simulink model "PSO_BON"  (R2019b)
settings: Solver=VariableStepAuto  StartTime=0.0  StopTime=0.2  RelTol=1e-5
undefined symbols (not defined in the file): sigbuilder_block
libraries: powerlib x164, re_lib x96, powerlib_meascontrol x9
(part 6 of 6)

== matlab function PSO_BON/Variant PSO/MATLAB Function1 ==
  settings: updateMethod=DISCRETE  sampleTime=1e-4
  data: Vpv input; Duty output; Ipv input
function Duty = PSO_SSR(Vpv,Ipv)
coder.extrinsic('rand')
coder.extrinsic('format long')

persistent Npart_3 v_3 iter_3 count_Part_3 count_3 pos_3 fitness_3 fitnessPbest_3 Pbest_3 fitnessGbest_3 fitnessGworst_3 Gbest_3 Gworst_3 count_conv_3 reinit_3 Duty_Init_3;
maxiter = 10000000;                                                         % Nombre d'itération

% Définition de l'espace de recherche
% ------------------------------------
duty_cl_min = 0.1;                                                          % Valeur minimale du rapport cyclique
duty_cl_max = 0.9;                                                          % Valeur maximale du rapport cyclique

% Tolérance de la puissance
% ------------------------------------
tolerance = 0.01;                                                           % Tolerance de la puissance en sortie

% Initialisation des vitesses des particules
% -------------------------------------------
if(isempty(Npart_3))
    Npart_3 = 10;
end
if(isempty(v_3))
    v_3 = zeros(Npart_3,1);
end

% Initialisation des positions des particules
% -------------------------------------------

% hybrid initialisation
% ---------------------  
if(isempty(pos_3))                                                          % Si la position des particules est inexistant
    r = zeros(Npart_3,1);
    r = rand(Npart_3,1);
    pos_3 = zeros(Npart_3,1);
    for i = 1:Npart_3-2
        Min = duty_cl_min + (i-1)*(duty_cl_max-duty_cl_min)/(Npart_3-2);
        Max = Min + (duty_cl_max-duty_cl_min)/(Npart_3-2);
        pos_3(i+1) = Min + r(i)*(Max-Min);
    end
    pos_3(1) = duty_cl_min;
    pos_3(Npart_3) = duty_cl_max;
end

% % Uniform initialisation
% % ----------------------  
% if(isempty(pos_3))                                                          % Si la position des particules est inexistant
%     pos_3 = zeros(Npart_3,1);
%     for i = 1:Npart_3-2
%         pos_3(i+1) = duty_cl_min + ((duty_cl_max-duty_cl_min)*(i-1))/(Npart_3-1);
%     end
%     pos_3(1) = duty_cl_min;
%     pos_3(Npart_3) = duty_cl_max;
% end
% 
% % Random initialisation
% % ---------------------  
% if(isempty(pos_3))                                                          % Si la position des particules est inexistant
%     pos_3 = zeros(Npart_3,1);
%     for i = 1:Npart_3-2
%         pos_3(i+1) = duty_cl_min + rand(1)*(duty_cl_max-duty_cl_min);
%     end
%     pos_3(1) = duty_cl_min;
%     pos_3(Npart_3) = duty_cl_max;
% end

% pos
% Initialisation des parametres persitents
% -------------------------------------------------
if(isempty(iter_3))       % Si le numéro de l'iteration est inexistant fixe à 1
    iter_3 = 1;
end
if(isempty(fitness_3))    % Si la fonction cout des particules est inexistant
    fitness_3 = zeros(Npart_3,1);
end
if(isempty(fitnessPbest_3))   % Si les fonctions couts des meilleures positions des particules est inexistant
    fitnessPbest_3 = zeros(Npart_3,1);
end
if(isempty(Pbest_3))      % Si les meilleures positions des particules est inexistant
    Pbest_3 = zeros(Npart_3,1);
end
if(isempty(Gbest_3))      % Si la meilleure position de l'éssain est inexistant
    Gbest_3 = zeros(maxiter,1);
end
if(isempty(Gworst_3))      % Si la meilleure position de l'éssain est inexistant
    Gworst_3 = zeros(maxiter,1);
end
if(isempty(fitnessGbest_3))   % Si la fonction cout de la meilleure position de l'éssain est inexistant
    fitnessGbest_3 = zeros(maxiter,1);
end
if(isempty(fitnessGworst_3))   % Si la fonction cout de la meilleure position de l'éssain est inexistant
    fitnessGworst_3 = zeros(maxiter,1);
end
if(isempty(count_Part_3)) % Si le compteur de particule est inexistant
    count_Part_3 = 1;
end
if(isempty(count_conv_3)) % Si le compteur de particule convergente est inexistant
    count_conv_3 = zeros(Npart_3,1);
end
if(isempty(reinit_3))   % Si le coefficeint de reinitialisation est inexistant
    reinit_3 = 0;
end
if(isempty(Duty_Init_3))
    Duty_Init_3 = 0;
end
if(isempty(count_3))      % Si le compteur du régime transitoire est inexistant
    count_3 = 1;
end


% Evaluation des particules initiales
% -------------------------------------------------

%% phase transitoire d'évaluation d'une particule
% -------------------------------------------------
if (count_3 >= 1 && count_3 <= 20)
    Duty = pos_3(count_Part_3);
    count_3 = count_3 + 1;

    %% En cas de convergence
    % ---------------------------------------------
    if (reinit_3 == 1)  
        fitnessGbest_3(iter_3) = Vpv*Ipv;
        Duty = Duty_Init_3;
            if (abs(fitnessGbest_3(iter_3) - fitnessGbest_3(iter_3-1)) < 1)
                count_3 = count_3 - 1;
                reinit_3 = 1;
            else
                reinit_3 = 0;
                Npart_3 = 10;
                r = zeros(Npart_3,1);
                r = rand(Npart_3,1);
                pos_3 = zeros(Npart_3,1);
                for i = 1:Npart_3-2
                    Min = duty_cl_min + (i-1)*(duty_cl_max-duty_cl_min)/(Npart_3-2);
                    Max = Min + (duty_cl_max-duty_cl_min)/(Npart_3-2);
                    pos_3(i+1) = Min + r(i)*(Max-Min);
                end
                pos_3(1) = duty_cl_min;
                pos_3(Npart_3) = duty_cl_max;
                iter_3 = 0;
                v_3 = zeros(Npart_3,1);
                fitness_3 = zeros(Npart_3,1);
                fitnessPbest_3 = zeros(Npart_3,1);
                Pbest_3 = zeros(Npart_3,1);
                Gbest_3 = zeros(maxiter,1);
                Gworst_3 = zeros(maxiter,1);
                fitnessGbest_3 = zeros(maxiter,1);
                fitnessGworst_3 = zeros(maxiter,1);
                count_Part_3 = 1;
                count_conv_3 = zeros(Npart_3,1);
                Duty_Init_3 = 0;
                count_3 = 1;
                iter_3 = iter_3 + 1;
            end 
    end
    return;
    
%%
Npart_3;
count_Part_3;
else
    Npart_3
    count_Part_3
    if(count_Part_3 <= (Npart_3 - 1))
        Duty = pos_3(count_Part_3 + 1);
    else
        Duty = pos_3(1);
    end
end
iter_3;
% pos
% fitness
% fitnessPbest

                        % Programme PSO principale ou se fait la
                        % mise à jour des Pbest, de Gbest, des vitesse et
                        % des positions des particules
                        % -------------------------------------------------
fitness_3(count_Part_3) = Vpv*Ipv;  % Fonction cout des particules
if (count_Part_3 <= (Npart_3 - 1))
    count_Part_3 = count_Part_3 + 1;
    count_3 = 2;
else
    nnn = 1;
    if (iter_3 == 1)
                        % Initialisation des Pbest
                        % -------------------------------------------------
            for i = 1:Npart_3
                Pbest_3(i) = pos_3(i);
                fitnessPbest_3(i) = fitness_3(i);
            end
                        % Détermination de la fonction cout maximale
                        % -------------------------------------------------
        maxFitnessPbest = 0;
        for j = 1:length(fitnessPbest_3)
            if fitnessPbest_3(j) > maxFitnessPbest
                maxFitnessPbest = fitnessPbest_3(j);
            end
        end
                        % Initialisation de Gbest
                        % -------------------------------------------------
        fitnessGbest_3(iter_3) = maxFitnessPbest;
            for k = 1:Npart_3
                if(fitnessGbest_3(iter_3) == fitnessPbest_3(k))
                    Gbest_3(iter_3) = Pbest_3(k);
                end
            end
    elseif (iter_3 >= 2 && iter_3 <= maxiter)
                        % Mise à jour des Pbest
                        % -------------------------------------------------
            for i = 1:Npart_3
                if (fitness_3(i) > fitnessPbest_3(i))
                    Pbest_3(i) = pos_3(i);
                    fitnessPbest_3(i) = fitness_3(i);
                end
            end
                        % Mise à jour de Gbest
                        % -------------------------------------------------
        maxFitnessPbest = 0;
        minFitnessPbest = 100000;
        for j = 1:length(fitnessPbest_3)
            if fitnessPbest_3(j) > maxFitnessPbest
                maxFitnessPbest = fitnessPbest_3(j);
            end
            if fitnessPbest_3(j) < minFitnessPbest
                minFitnessPbest = fitnessPbest_3(j);
            end
        end
        fitnessGbest_3(iter_3) = maxFitnessPbest;
        fitnessGworst_3(iter_3) = minFitnessPbest;
            nn = 0;
            for k=1:Npart_3
                if(fitnessGbest_3(iter_3) == fitnessPbest_3(k))
                    Gbest_3(iter_3) = Pbest_3(k);
                end
                if(fitnessGworst_3(iter_3) == fitnessPbest_3(k))
                    Gworst_3(iter_3) = Pbest_3(k);
                    nn = k;
                end
            end
        nn;
        if (iter_3 > 2)
            if (Npart_3 >= 2)
                Npart_3 = Npart_3 - nnn;
                Pbest_3(nn) = [];
                pos_3(nn) = [];
                fitness_3(nn) = [];
                fitnessPbest_3(nn) = [];
                v_3(nn) = [];
                count_conv_3(nn) = [];
                nnn = nnn + 1;
            end
        end
    end
    pos_3;
    count_Part_3;
    iter_3;
    Npart_3
    count_Part_3
                        % Test de convergence
                        % -------------------------------------------------
        for i = 1:Npart_3
            if ((fitnessGbest_3(iter_3) - fitnessPbest_3(i)) < tolerance)
                if ((Gbest_3(iter_3) - pos_3(i)) < 0.0001)
                    count_conv_3(i) = 1;
                end
            end
        end
    n = sum(count_conv_3);
    if (n == Npart_3)
        reinit_3 = 1;
        Duty_Init_3 = Gbest_3(iter_3);
    else
        count_conv_3 = zeros(Npart_3,1);
    end
                        % Mise à jour des positions et des vitesses des
                        % particules
                        % -------------------------------------------------
        for i = 1:Npart_3
            v_3(i) = updatevelocity(v_3(i),Pbest_3(i),pos_3(i),Gbest_3(iter_3),iter_3,50);
            pos_3(i) = updateduty(pos_3(i),v_3(i));
            if (pos_3(i) > duty_cl_max)
                pos_3(i) = duty_cl_max;
            end
            if (pos_3(i) < duty_cl_min)
                pos_3(i) = duty_cl_min;
            end
        end
                        % Mise à jour des positions et des vitesses
                        % -------------------------------------------------

                        % Contraindre la position mise à jour dans
                        % l'intervale de recherche
                        % -------------------------------------------------
    Duty = pos_3(1);
    count_Part_3 = 1;
    count_3 = 2;
    iter_3 = iter_3 + 1;
    if iter_3 > maxiter
        iter_3 = maxiter;
    end
end
end

function vfinal=updatevelocity(velocity,pobest,d,gwbest,Iter, Maxiter)

w1 = 0.1;
w2 = 0.2;
w = ((w1 - w2)*(Maxiter - Iter))/Maxiter + w2;

c1f = 0.0015;       % Personal Learning Coefficient
c1i = 1;         % Global Learning Coefficient
c1 = ((c1f - c1i)*(Iter))/Maxiter + c1i;

c2f = 1.4;       % Personal Learning Coefficient
c2i = 0.3;         % Global Learning Coefficient
c2 = ((c2f - c2i)*(Iter))/Maxiter + c2i;

vfinal = (w*velocity)+(c1*rand(1)*(pobest-d))+(c2*rand(1)*(gwbest-d));
% vfinal = (w*velocity)+beta*(gwbest-d);
end
function dfinal=updateduty(d,velocity)
dup=d+velocity;
if(dup>0.9)
    dfinal=0.9;
elseif(dup<0.1)
    dfinal=0.1;
else
    dfinal=dup;
end
end

== matlab function PSO_BON/Dynamique PSOO/MATLAB Function1 ==
  settings: updateMethod=DISCRETE  sampleTime=1e-4
  data: Vpv input; D output; Ipv input
function D = PSO(Vpv,Ipv)
%#codegen
persistent u;
persistent dcurrent;
persistent pbest;
persistent p;
persistent dc;
persistent v;
persistent counter;
persistent gbest;
persistent K;
Npart = 10;
maxIte = 15;
if(isempty(counter))
    counter=0;
end
if(isempty(dcurrent))
    dcurrent=0.5;
end
if(isempty(gbest))
    gbest=0.5;
end
if(isempty(p))
    p=zeros(Npart,1);
end
if(isempty(K))
    K=0;
end
if(isempty(v))
    v=zeros(Npart,1);
end

if(isempty(pbest))
    pbest=zeros(Npart,1);
end
if(isempty(u))
    u=0;
end
if(isempty(dc))
    dc=zeros(Npart,1);
    dc(1)=0;
    dc(2)=0.1;
    dc(3)=0.2;
    dc(4)=0.3;
    dc(5)=0.4;
    dc(6)=0.5;
    dc(7)=0.6;
    dc(8)=0.7;
    dc(9)=0.8;
    dc(10)=0.9;
end
if(counter>=1 && counter<20)
    D=dcurrent;
    counter=counter+1;
    return;
end
counter=0;

if(u>=1 && u<=Npart)
    if((Vpv*Ipv)>p(u))
        p(u)=Vpv*Ipv;
        pbest(u)=dcurrent;
    end
end
u=u+1;
if(u==Npart+2)
    u=1;
end
if(u==1)
    D=dc(u);
    dcurrent=D;
    counter=1;
    return;
elseif(u==2)
    D=dc(u);
    dcurrent=D;
    counter=1;
    return;
elseif(u==3)
    D=dc(u);
    dcurrent=D;
    counter=1;
    return;
elseif(u==4)
    D=dc(u);
    dcurrent=D;
    counter=1;
    return;
elseif(u==5)
    D=dc(u);
    dcurrent=D;
    counter=1;
    return;
elseif(u==6)
    D=dc(u);
    dcurrent=D;
    counter=1;
    return;
elseif(u==7)
    D=dc(u);
    dcurrent=D;
    counter=1;
    return;
elseif(u==8)
    D=dc(u);
    dcurrent=D;
    counter=1;
    return;
elseif(u==9)
    D=dc(u);
    dcurrent=D;
    counter=1;
    return;
elseif(u==10)
    D=dc(u);
    dcurrent=D;
    counter=1;
    return;
elseif(u==Npart+1)
    [m,i]=max(p);
    gbest=pbest(i);
    D=gbest;
    dcurrent=D;
    counter=1;
    K = K + 1;
    %update velocity and duty cycle
    v(1)=updatevelocity(v(1),pbest(1),dc(1),gbest,maxIte,K)
    v(2)=updatevelocity(v(2),pbest(2),dc(2),gbest,maxIte,K)
    v(3)=updatevelocity(v(3),pbest(3),dc(3),gbest,maxIte,K)
    v(4)=updatevelocity(v(4),pbest(4),dc(4),gbest,maxIte,K)
    v(5)=updatevelocity(v(5),pbest(5),dc(5),gbest,maxIte,K)
    v(6)=updatevelocity(v(6),pbest(6),dc(6),gbest,maxIte,K)
    v(7)=updatevelocity(v(7),pbest(7),dc(7),gbest,maxIte,K)
    v(8)=updatevelocity(v(8),pbest(8),dc(8),gbest,maxIte,K)
    v(9)=updatevelocity(v(9),pbest(9),dc(9),gbest,maxIte,K)
    v(10)=updatevelocity(v(10),pbest(10),dc(10),gbest,maxIte,K)
    %update duty cycle
    dc(1)=updateduty(dc(1),v(1))
    dc(2)=updateduty(dc(2),v(2))
    dc(3)=updateduty(dc(3),v(3))
    dc(4)=updateduty(dc(4),v(4))
    dc(5)=updateduty(dc(5),v(5))
    dc(6)=updateduty(dc(6),v(6))
    dc(7)=updateduty(dc(7),v(7))
    dc(8)=updateduty(dc(8),v(8))
    dc(9)=updateduty(dc(9),v(9))
    dc(10)=updateduty(dc(10),v(10))
    
    return;
    
else
    u
    y='hello'
    D=0.1
    
end


end
function vfinal=updatevelocity(velocity,pobest,d,gwbest,maxIte,K)
% PSO Parameters
w=0.4;
c1=1.2;       % Personal Learning Coefficient
c2=2;         % Global Learning Coefficient
beta = 1.5;
wmax=1; wmin=0.1; %w=0.5; 
c1max=1.2;  c1min=1; c2max=1.6;  c2min=1;
w=wmax-(wmax-wmin)/maxIte*K;
c1=c1max-(c1max-c1min)/maxIte*K;
c2=c2max-(c2max-c2min)/maxIte*K;
% % Constriction Coefficients
% phi1=2.05;
% phi2=2.05;
% phi=phi1+phi2;
% chi=2/(phi-2+sqrt(phi^2-4*phi));
% w=chi;          % Inertia Weight
% wdamp=1;        % Inertia Weight Damping Ratio
% c1=chi*phi1;    % Personal Learning Coefficient
% c2=chi*phi2;    % Global Learning Coefficient
vfinal = (w*velocity)+(c1*rand(1)*(pobest-d))+(c2*rand(1)*(gwbest-d));
% vfinal = (w*velocity)+beta*(gwbest-d);
end
function dfinal=updateduty(d,velocity)
dup=d+velocity;
if(dup>0.9)
    dfinal=0.9;
elseif(dup<0.1)
    dfinal=0.1;
else
    dfinal=dup;
end
end

== matlab function PSO_BON/P&O/MATLAB Function1 ==
  settings: updateMethod=DISCRETE  sampleTime=1e-4
  data: Vpv input; D output; Ipv input
function D = PSO_Mod(Vpv,Ipv)
coder.extrinsic('rand')
coder.extrinsic('format long')

persistent iter count_Part count pos fitness fitnessPbest Pbest fitnessGbest Gbest count_conv reinit Duty_Init Vpos Ipos;
persistent Vgbest Igbest Vposbest Iposbest;
Npart = 5;              % Nombre de particules de l'éssain
maxiter = 10000000;           % Nombre d'itération
delta = 0.05;
% Espace de recherche
% ------------------------------------
duty_cl_min = 0.1;      % Valeur minimale du rapport cyclique
duty_cl_max = 0.9;      % Valeur maximale du rapport cyclique

% Tolérance de la puissance
% ------------------------------------
tolerance = 1;          % Tolerance de la puissance en sortie

% Initialisation des positions des particules
% ------------------------------------
r = zeros(Npart,1);     % génération d'un vecteur de nombre aléatoire compris entre 0 et 1
r = rand(Npart,1);      
if(isempty(pos))        % Si la position des particules est inexistant
    pos = zeros(Npart,1);
%     for i = 1:Npart
%         pos(i) = duty_cl_min + ((duty_cl_max-duty_cl_min)*(i-1))/(Npart-1);
% %         pos(i) = duty_cl_min + r(i)*(duty_cl_max-duty_cl_min);
%     end
    
    for i = 1:Npart-2
        Min = duty_cl_min + (i-1)*(duty_cl_max-duty_cl_min)/(Npart-2);
        Max = Min + (duty_cl_max-duty_cl_min)/(Npart-2);
        pos(i+1) = Min + r(i)*(Max-Min);
    end
    pos(1) = duty_cl_min;
    pos(Npart) = duty_cl_max;
    Pp = pos;
end

% Initialisation des parametres persitents
% -------------------------------------------------
if(isempty(iter))       % Si le numéro de l'iteration est inexistant fixe à 1
    iter = 1;
end
if(isempty(fitness))    % Si la fonction cout des particules est inexistant
    fitness = zeros(Npart,1);
end
if(isempty(Vpos))    % Si la fonction cout des particules est inexistant
    Vpos = zeros(Npart,1);
end
if(isempty(Ipos))    % Si la fonction cout des particules est inexistant
    Ipos = zeros(Npart,1);
end
if(isempty(fitnessPbest))   % Si les fonctions couts des meilleures positions des particules est inexistant
    fitnessPbest = zeros(Npart,1);
end
if(isempty(Pbest))      % Si les meilleures positions des particules est inexistant
    Pbest = zeros(Npart,1);
    P = Pbest;
end
if(isempty(Vposbest))      % Si les meilleures positions des particules est inexistant
    Vposbest = zeros(Npart,1);
end
if(isempty(Iposbest))      % Si les meilleures positions des particules est inexistant
    Iposbest = zeros(Npart,1);
end
if(isempty(Gbest))      % Si la meilleure position de l'éssain est inexistant
    Gbest = zeros(maxiter,1);
end
if(isempty(fitnessGbest))   % Si la fonction cout de la meilleure position de l'éssain est inexistant
    fitnessGbest = zeros(maxiter,1);
end
if(isempty(Vgbest))   % Si la fonction cout de la meilleure position de l'éssain est inexistant
    Vgbest = zeros(maxiter,1);
end
if(isempty(Igbest))   % Si la fonction cout de la meilleure position de l'éssain est inexistant
    Igbest = zeros(maxiter,1);
end
if(isempty(count_Part)) % Si le compteur de particule est inexistant
    count_Part = 1;
end
if(isempty(count_conv)) % Si le compteur de particule convergente est inexistant
    count_conv = zeros(Npart,1);
end
if(isempty(reinit))   % Si le coefficeint de reinitialisation est inexistant
    reinit = 0;
end
if(isempty(Duty_Init))
    Duty_Init = 0;
end
if(isempty(count))      % Si le compteur du régime transitoire est inexistant
    count = 1;
end

% Evaluation des particules initiales
% -------------------------------------------------
if (count >= 1 && count <= 20)
    D = pos(count_Part);
    G = Duty_Init;
    P = Pbest;
    Pp = pos;
    count = count + 1;            % Incrémenter
    if (reinit == 1)
        D = Duty_Init;
        G = Duty_Init;
        P = Pbest;
        Pp = pos;
        count = count - 1;          % Décrémenter
    end
    return;
    
else
    if(count_Part <= (Npart - 1))
        D = pos(count_Part + 1);
        G = Gbest(iter);
        P = Pbest;
        Pp = pos;
    else
        D = pos(1);
        G = Gbest(iter);
        P = Pbest;
        Pp = pos;
    end
end
                        % Programme PSO principale ou se fait la
                        % mise à jour des Pbest, de Gbest, des vitesse et
                        % des positions des particules
                        % -------------------------------------------------
fitness(count_Part) = Vpv*Ipv;  % Fonction cout des particules
Vpos(count_Part) = Vpv;  % Fonction cout des particules
Ipos(count_Part) = Ipv;  % Fonction cout des particules
if (count_Part <= (Npart - 1))
    count_Part = count_Part + 1;
    count = 2;
else
    Pp = pos;
    if (iter == 1)
                        % Initialisation des Pbest
                        % -------------------------------------------------
        for i = 1:Npart
            Pbest(i) = pos(i);
            fitnessPbest(i) = fitness(i);
            Vposbest(i) = Vpos(i);
            Iposbest(i) = Ipos(i);
        end
        P = Pbest;
        Pp = pos;
                        % Détermination de la fonction cout maximale
                        % -------------------------------------------------
        maxFitnessPbest = 0;
        for j = 1:length(fitnessPbest)
            if fitnessPbest(j) > maxFitnessPbest
                maxFitnessPbest = fitnessPbest(j);
            end
        end
                        % Initialisation de Gbest
                        % -------------------------------------------------
        fitnessGbest(iter) = maxFitnessPbest;
        for k = 1:Npart
            if(fitnessGbest(iter) == fitnessPbest(k))
                Gbest(iter) = Pbest(k);
                Vgbest(iter) = Vposbest(k);
                Igbest(iter) = Iposbest(k);
            end
        end
    elseif (iter >= 2 && iter <= maxiter)
                        % Mise à jour des Pbest
                        % -------------------------------------------------
        for i = 1:Npart
            if (fitness(i) > fitnessPbest(i))
                Pbest(i) = pos(i);
                fitnessPbest(i) = fitness(i);
                Vposbest(i) = Vpos(i);
                Iposbest(i) = Ipos(i);
            end
        end
        P = Pbest;
        Pp = pos;
                        % Mise à jour de Gbest
                        % -------------------------------------------------
        maxFitnessPbest = 0;
        for j = 1:length(fitnessPbest)
            if fitnessPbest(j) > maxFitnessPbest
                maxFitnessPbest = fitnessPbest(j);
            end
        end
        fitnessGbest(iter) = maxFitnessPbest;
        for k=1:Npart
            if(fitnessGbest(iter) == fitnessPbest(k))
                Gbest(iter) = Pbest(k);
                Vgbest(iter) = Vposbest(k);
                Igbest(iter) = Iposbest(k);
            end
        end
    end
    G = Gbest(iter);
                       % Test de convergence
                        % -------------------------------------------------
    for i = 1:Npart
        if ((fitnessGbest(iter) - fitnessPbest(i)) < tolerance)
            count_conv(i) = 1;
        end
    end
    n = sum(count_conv);
    if (n == Npart)
        reinit = 1;
        Duty_Init = Gbest(iter);
        G = Gbest(iter);
    else
        count_conv = zeros(Npart,1);
        G = Gbest(iter);
    end
                        % Mise à jour des positions et des vitesses des
                        % particules
                        % -------------------------------------------------
    for i = 1:Npart
                        % Mise à jour des positions sur le principe de la
                        % dichotomie
                        % -------------------------------------------------
            dV = Vpos(i) - Vgbest(iter);
%             dI = Ipos(i) - Igbest(iter);
            if dV == 0
%                 if dI == 0
                    pos(i) = pos(i);
%                 else
%                     if dI > 0
%                         pos(i) = pos(i) - delta;
%                     else
%                         pos(i) = pos(i) + delta;
%                     end
%                 end
            else
                if dV < 0
%                     pos(i) = pos(i);
%                 else
%                     if dI/dV < -Ipos(i)/Vpos(i)
                        pos(i) = pos(i) - 0.25*Gbest(iter);
                    else
                        pos(i) = pos(i) + 0.25*Gbest(iter);
                    end
                end
%             end
%     end
                        % Contraindre la position mise à jour dans
                        % l'intervale de recherche
                        % -------------------------------------------------
        if (pos(i) > duty_cl_max)
            pos(i) = duty_cl_max;
        end
        if (pos(i) < duty_cl_min)
            pos(i) = duty_cl_min;
        end
    end
    D = pos(1);
    G = Gbest(iter);
    P = Pbest;
    Pp = pos
    count_Part = 1;
    count = 2;
    iter = iter + 1;
    if iter > maxiter
        iter = maxiter;
    end
end
end

== matlab function PSO_BON/Free-Parameter PSO/MATLAB Function2 ==
  settings: updateMethod=DISCRETE  sampleTime=1e-4
  data: Vpv input; D output; Ipv input
function D  = PSO_Mod(Vpv,Ipv)
coder.extrinsic('rand')
coder.extrinsic('format long')

%% Déclaration et initialisation des variables
% --------------------------------------------

persistent iter_1 count_Part_1 count_1 pos_1 fitness_1 fitnessPbest_1 Pbest_1 fitnessGbest_1 Gbest_1 count_conv_1 reinit_1 Duty_Init_1;
Npart = 10;                                                                 % Nombre de particules de l'éssain
maxiter = 10000000;                                                         % Nombre d'itération

% Définition de l'espace de recherche
% -----------------------------------
duty_cl_min = 0.1;                                                          % Valeur minimale du rapport cyclique
duty_cl_max = 0.9;                                                          % Valeur maximale du rapport cyclique

% Tolérance de la puissance
% -------------------------
tolerance = 1;                                                           % Tolerance de la puissance en sortie

% Initialisation des positions des particules
% -------------------------------------------

% hybrid initialisation
% ---------------------  
r = zeros(Npart,1);
r = rand(Npart,1);
if(isempty(pos_1))                                                          % Si la position des particules est inexistant
    pos_1 = zeros(Npart,1);
    for i = 1:Npart-2
        Min = duty_cl_min + (i-1)*(duty_cl_max-duty_cl_min)/(Npart-2);
        Max = Min + (duty_cl_max-duty_cl_min)/(Npart-2);
        pos_1(i+1) = Min + r(i)*(Max-Min);
    end
    pos_1(1) = duty_cl_min;
    pos_1(Npart) = duty_cl_max;
end

% % Uniform initialisation
% % ----------------------  
% if(isempty(pos_1))                                                          % Si la position des particules est inexistant
%     pos_1 = zeros(Npart,1);
%     for i = 1:Npart-2
%         pos_1(i+1) = duty_cl_min + ((duty_cl_max-duty_cl_min)*(i-1))/(Npart-1);
%     end
%     pos_1(1) = duty_cl_min;
%     pos_1(Npart) = duty_cl_max;
% end
% 
% % Random initialisation
% % ---------------------  
% if(isempty(pos_1))                                                          % Si la position des particules est inexistant
%     pos_1 = zeros(Npart,1);
%     for i = 1:Npart-2
%         pos_1(i+1) = duty_cl_min + rand(1)*(duty_cl_max-duty_cl_min);
%     end
%     pos_1(1) = duty_cl_min;
%     pos_1(Npart) = duty_cl_max;
% end
    
% Initialisation des parametres persitents
% ----------------------------------------
if(isempty(iter_1))                                                         % Si le numéro de l'iteration est inexistant fixer à 1
    iter_1 = 1;
end

if(isempty(fitness_1))                                                      % Si la fonction cout des particules est inexistante
    fitness_1 = zeros(Npart,1);
end

if(isempty(fitnessPbest_1))                                                 % Si les fonctions couts des meilleures positions des particules sont inexistantes
    fitnessPbest_1 = zeros(Npart,1);
end

if(isempty(Pbest_1))                                                        % Si les meilleures positions des particules sont inexistantes
    Pbest_1 = zeros(Npart,1);
end

if(isempty(Gbest_1))                                                        % Si la meilleure position de l'éssain est inexistante
    Gbest_1 = zeros(maxiter,1);
end

if(isempty(fitnessGbest_1))                                                 % Si la fonction cout de la meilleure position de l'éssain est inexistante
    fitnessGbest_1 = zeros(maxiter,1);
end

if(isempty(count_Part_1))                                                   % Si le compteur de particule est inexistant
    count_Part_1 = 1;
end
if(isempty(count_conv_1))                                                   % Si le compteur de particule convergente est inexistant
    count_conv_1 = zeros(Npart,1);
end

if(isempty(reinit_1))                                                       % Si le coefficeint de reinitialisation est inexistant
    reinit_1 = 0;
end

if(isempty(Duty_Init_1))                                                    % Si le rapport cyclique initial est inexistant
    Duty_Init_1 = 0;
end

if(isempty(count_1))                                                        % Si le compteur du régime transitoire est inexistant
    count_1 = 1;
end

%% Evaluation des particules initiales
% ------------------------------------

% phase transitoire d'évaluation de chacune des particules
% --------------------------------------------------------
if (count_1 >= 1 && count_1 <= 20)
    D = pos_1(count_Part_1);
    count_1 = count_1 + 1;

    % En cas de convergence
    % ---------------------
	if (reinit_1 == 1)  
        fitnessGbest_1(iter_1) = Vpv*Ipv;
        D = Duty_Init_1;
        if (abs(fitnessGbest_1(iter_1) - fitnessGbest_1(iter_1-1)) < 1)
            count_1 = count_1 - 1;
           	reinit_1 = 1;
        else
	
          	reinit_1 = 0;
            % initialisation
            % --------------
            r = zeros(Npart,1);
            r = rand(Npart,1);
            pos_1 = zeros(Npart,1);
            for i = 1:Npart-2
                Min = duty_cl_min + (i-1)*(duty_cl_max-duty_cl_min)/(Npart-2);
                Max = Min + (duty_cl_max-duty_cl_min)/(Npart-2);
                pos_1(i+1) = Min + r(i)*(Max-Min);
            end
            pos_1(1) = duty_cl_min;
            pos_1(Npart) = duty_cl_max;
           	iter_1 = 0;
          	fitness_1 = zeros(Npart,1);
           	fitnessPbest_1 = zeros(Npart,1);
          	Pbest_1 = zeros(Npart,1);
          	Gbest_1 = zeros(maxiter,1);
          	fitnessGbest_1 = zeros(maxiter,1);
           	count_Part_1 = 1;
           	count_conv_1 = zeros(Npart,1);
          	Duty_Init_1 = 0;
           	count_1 = 1;
            iter_1 = iter_1 + 1;
        end
        
 	end
    return;

else
    pos_1
    if(count_Part_1 <= (Npart - 1))
        D = pos_1(count_Part_1 + 1);
    else
        D = pos_1(1);
    end
end

%% Mises à jour des Pbest et Gbest
                        % Programme PSO principale ou se fait la
                        % mise à jour des Pbest, de Gbest, des vitesse et
                        % des positions des particules
                        % -------------------------------------------------
fitness_1(count_Part_1) = Vpv*Ipv;  % Fonction cout des particules
if (count_Part_1 <= (Npart - 1))
    count_Part_1 = count_Part_1 + 1;
    count_1 = 2;
else
    if (iter_1 == 1)
                        % Initialisation des Pbest
                        % -------------------------------------------------
        for i = 1:Npart
            Pbest_1(i) = pos_1(i);
            fitnessPbest_1(i) = fitness_1(i);
        end
                        % Détermination de la fonction cout maximale
                        % -------------------------------------------------
        maxFitnessPbest = 0;
        for j = 1:length(fitnessPbest_1)
            if fitnessPbest_1(j) > maxFitnessPbest
                maxFitnessPbest = fitnessPbest_1(j);
            end
        end
                        % Initialisation de Gbest
                        % -------------------------------------------------
        fitnessGbest_1(iter_1) = maxFitnessPbest;
        for k = 1:Npart
            if(fitnessGbest_1(iter_1) == fitnessPbest_1(k))
                Gbest_1(iter_1) = Pbest_1(k);
            end
        end
    elseif (iter_1 >= 2 && iter_1 <= maxiter)
                        % Mise à jour des Pbest
                        % -------------------------------------------------
        for i = 1:Npart
            if (fitness_1(i) > fitnessPbest_1(i))
                Pbest_1(i) = pos_1(i);
                fitnessPbest_1(i) = fitness_1(i);
            end
        end
                        % Mise à jour de Gbest
                        % -------------------------------------------------
        maxFitnessPbest = 0;
        for j = 1:length(fitnessPbest_1)
            if fitnessPbest_1(j) > maxFitnessPbest
                maxFitnessPbest = fitnessPbest_1(j);
            end
        end
        fitnessGbest_1(iter_1) = maxFitnessPbest;
        for k=1:Npart
            if(fitnessGbest_1(iter_1) == fitnessPbest_1(k))
                Gbest_1(iter_1) = Pbest_1(k);
            end
        end
    end
                        % Test de convergence
                        % -------------------------------------------------
%     for i = 1:Npart
%             if ((fitnessGbest_1(iter_1) - fitnessPbest_1(i)) < tolerance)
%                 if ((Gbest_1(iter_1) - pos_1(i)) < 0.0001)
%                     count_conv_1(i) = 1;
%                 end
%             end
%     end
    for i = 1:Npart
        if ((fitnessGbest_1(iter_1) - fitnessPbest_1(i)) < tolerance)
            count_conv_1(i) = 1;
        end
    end
    n = sum(count_conv_1);
    if (n == Npart)
        reinit_1 = 1;
        Duty_Init_1 = Gbest_1(iter_1);
    else
        count_conv_1 = zeros(Npart,1);
    end
                        % Mise à jour des positions sur le principe de la
                        % dichotomie
                        % -------------------------------------------------
    for i = 1:Npart
        pos_1(i) = (Gbest_1(iter_1)+pos_1(i))/2;
                        % Contraindre la position mise à jour dans
                        % l'intervale de recherche
                        % -------------------------------------------------
        if (pos_1(i) > duty_cl_max)
            pos_1(i) = duty_cl_max;
        end
        if (pos_1(i) < duty_cl_min)
            pos_1(i) = duty_cl_min;
        end
    end
    reinit_1
    pos_1
    D = pos_1(1);
    count_Part_1 = 1;
    count_1 = 2;
    iter_1 = iter_1 + 1;
    if iter_1 > maxiter
        iter_1 = maxiter;
    end
end
end
